simulink model "Detachable_Battery_Pack_V2"  (R2024a)
settings: Solver=VariableStepAuto  StartTime=0.0  StopTime=3600*2  RelTol=1e-3
libraries: fl_lib x5, nesl_utility x3, simulink x2, batt_lib x1, BatteryPack_UR18650ZTA_lib x1
settings Model: Creator=MANSY  LastModifiedBy=MANSY

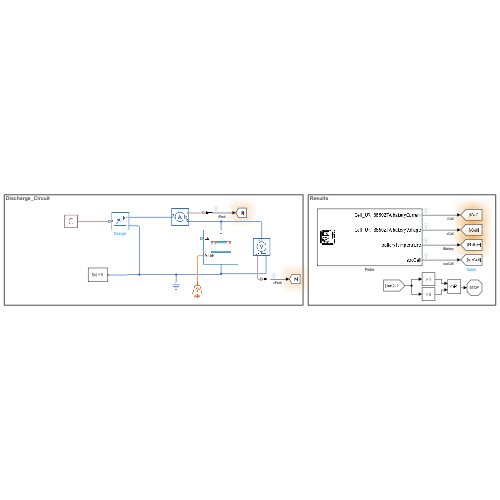
[thumbnail: Simulink's stored preview of the top-level diagram]
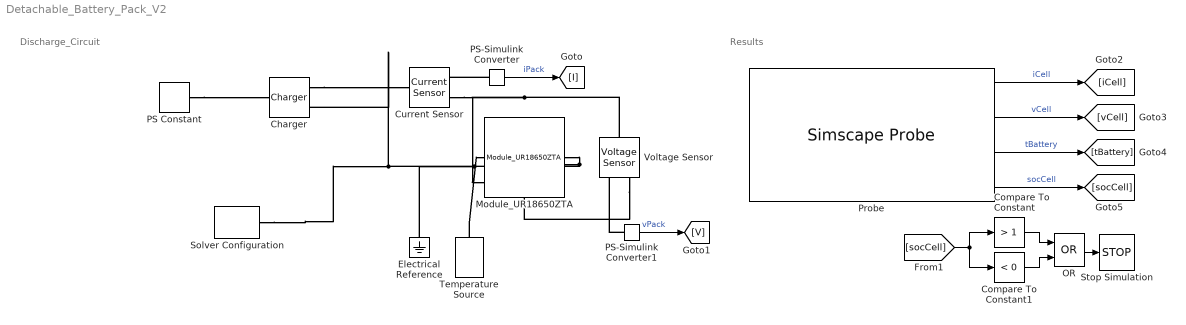
== system Detachable_Battery_Pack_V2 ==
  note: Results
  note: Discharge_Circuit
  Charger : batt_lib/Cyclers/Charger  charging_current=10.6 A  voltage_threshold=21 V  charging_voltage=21 V  current_threshold=0.5 A
      settings: InternalSimscapePortConfiguration="{\"Bottom\":[],\"Left\":[{\"id\":\"trigger\",\"label\":\"t\",\"type\":\"input\"}],\"Right\":[{\"id\":\"p\",\"label\":\"+\",\"type\":\"foundation.electrical.electrical\"},{\"id\":\"n\",\"label\":\"-\",\"type\":\"foundation.electrical.electrical\"}],\"Top\":[]}"
  Compare To Constant : simulink/Logic and Bit Operations/Compare To Constant  relop=>  const=1  OutDataTypeStr=boolean
  Compare To Constant1 : simulink/Logic and Bit Operations/Compare To Constant  relop=<  const=0  OutDataTypeStr=boolean
  Current Sensor : fl_lib/Electrical/Electrical Sensors/Current Sensor
  Electrical Reference : fl_lib/Electrical/Electrical Elements/Electrical Reference
  Module_UR18650ZTA : BatteryPack_UR18650ZTA_lib/Module_UR18650ZTA  BatteryCapacityCell=2.65 A*hr  ExtrapolationMethodCell=simscape.enum.extrapolation.linear  SOCBreakpointsCell=[0, .01, .02, .03, .04, .05, .06, .07, .08, .09, .1, .11, .12, .13, .14, .15, .16, .17, .18, .19, .2, .21, .22, .23, .24, .25, .26, .27, .28, .29, .3, .31, .32, .33, .34, .35, .36, .37, .38, .39, .4, .41, .42, .43, .44, .45, .46, .47, .48, .49, .5, .51, .52, .53, .54, .55, .56, .57, .58, .59, .6, .61, .62, .63, .64, .65, .66, .67, .68, .69, .7, .71, .72, .73, .74, .75, .76, .77, .78, .79, .8, .81, .82, .83, .84, .85, .86, .87, .88, .89, .9, .91, .92, .93, .94, .95, .96, .97, .98, .99, 1]  TemperatureBreakpointsCell=[0, 25, 40, 60] degC  OpenCircuitVoltageThermalCell=[3.04339, 3.04339, 3.04339, 3.04339; 3.19969, 3.19969, 3.19969, 3.19969; 3.32733, 3.32733, 3.32733, 3.32733; 3.41897, 3.41897, 3.41897, 3.41897; 3.47789, 3.47789, 3.47789, 3.47789; 3.5189, 3.5189, 3.5189, 3.5189; 3.54757, 3.54757, 3.54757, 3.54757; 3.56926, 3.56926, 3.56926, 3.56926; 3.58543, 3.58543, 3.58543, 3.58543; 3.59715, 3.59715, 3.59715, 3.59715; 3.60656, 3.60656, 3.60656, 3.60656; 3.61458, 3.61458, 3.61458, 3.61458; 3.62125, 3.62125, 3.62125, 3.62125; 3.62859, 3.62859, 3.62859, 3.62859; 3.63585, 3.63585, 3.63585, 3.63585; 3.64117, 3.64117, 3.64117, 3.64117; 3.64677, 3.64677, 3.64677, 3.64677; 3.65281, 3.65281, 3.65281, 3.65281; 3.65754, 3.65754, 3.65754, 3.65754; 3.6622, 3.6622, 3.6622, 3.6622; 3.66686, 3.66686, 3.66686, 3.66686; 3.67118, 3.67118, 3.67118, 3.67118; 3.67547, 3.67547, 3.67547, 3.67547; 3.67953, 3.67953, 3.67953, 3.67953; 3.68333, 3.68333, 3.68333, 3.68333; 3.68679, 3.68679, 3.68679, 3.68679; 3.68929, 3.68929, 3.68929, 3.68929; 3.69163, 3.69163, 3.69163, 3.69163; 3.69398, 3.69398, 3.69398, 3.69398; 3.69633, 3.69633, 3.69633, 3.69633; 3.69868, 3.69868, 3.69868, 3.69868; 3.70108, 3.70108, 3.70108, 3.70108; 3.7035, 3.7035, 3.7035, 3.7035; 3.70592, 3.70592, 3.70592, 3.70592; 3.70834, 3.70834, 3.70834, 3.70834; 3.71076, 3.71076, 3.71076, 3.71076; 3.71334, 3.71334, 3.71334, 3.71334; 3.71599, 3.71599, 3.71599, 3.71599; 3.71889, 3.71889, 3.71889, 3.71889; 3.72198, 3.72198, 3.72198, 3.72198; 3.72508, 3.72508, 3.72508, 3.72508; 3.72817, 3.72817, 3.72817, 3.72817; 3.73126, 3.73126, 3.73126, 3.73126; 3.73436, 3.73436, 3.73436, 3.73436; 3.73745, 3.73745, 3.73745, 3.73745; 3.74054, 3.74054, 3.74054, 3.74054; 3.74364, 3.74364, 3.74364, 3.74364; 3.74686, 3.74686, 3.74686, 3.74686; 3.75011, 3.75011, 3.75011, 3.75011; 3.75346, 3.75346, 3.75346, 3.75346; 3.75768, 3.75768, 3.75768, 3.75768; 3.7621, 3.7621, 3.7621, 3.7621; 3.76652, 3.76652, 3.76652, 3.76652; 3.77094, 3.77094, 3.77094, 3.77094; 3.77575, 3.77575, 3.77575, 3.77575; 3.78058, 3.78058, 3.78058, 3.78058; 3.78546, 3.78546, 3.78546, 3.78546; 3.79147, 3.79147, 3.79147, 3.79147; 3.79777, 3.79777, 3.79777, 3.79777; 3.80409, 3.80409, 3.80409, 3.80409; 3.8104, 3.8104, 3.8104, 3.8104; 3.81672, 3.81672, 3.81672, 3.81672; 3.82303, 3.82303, 3.82303, 3.82303; 3.82935, 3.82935, 3.82935, 3.82935; 3.83618, 3.83618, 3.83618, 3.83618; 3.84344, 3.84344, 3.84344, 3.84344; 3.8508, 3.8508, 3.8508, 3.8508; 3.85816, 3.85816, 3.85816, 3.85816; 3.86553, 3.86553, 3.86553, 3.86553; 3.87289, 3.87289, 3.87289, 3.87289; 3.88052, 3.88052, 3.88052, 3.88052; 3.88833, 3.88833, 3.88833, 3.88833; 3.89603, 3.89603, 3.89603, 3.89603; 3.90423, 3.90423, 3.90423, 3.90423; 3.91256, 3.91256, 3.91256, 3.91256; 3.92124, 3.92124, 3.92124, 3.92124; 3.93029, 3.93029, 3.93029, 3.93029; 3.93933, 3.93933, 3.93933, 3.93933; 3.94837, 3.94837, 3.94837, 3.94837; 3.95788, 3.95788, 3.95788, 3.95788; 3.96788, 3.96788, 3.96788, 3.96788; 3.97854, 3.97854, 3.97854, 3.97854; 3.98931, 3.98931, 3.98931, 3.98931; 4.00008, 4.00008, 4.00008, 4.00008; 4.01149, 4.01149, 4.01149, 4.01149; 4.02304, 4.02304, 4.02304, 4.02304; 4.03459, 4.03459, 4.03459, 4.03459; 4.04614, 4.04614, 4.04614, 4.04614; 4.05768, 4.05768, 4.05768, 4.05768; 4.06947, 4.06947, 4.06947, 4.06947; 4.08184, 4.08184, 4.08184, 4.08184; 4.09422, 4.09422, 4.09422, 4.09422; 4.1067, 4.1067, 4.1067, 4.1067; 4.11982, 4.11982, 4.11982, 4.11982; 4.1326, 4.1326, 4.1326, 4.1326; 4.14615, 4.14615, 4.14615, 4.14615; 4.15754, 4.15754, 4.15754, 4.15754; 4.16699, 4.16699, 4.16699, 4.16699; 4.17222, 4.17222, 4.17222, 4.17222; 4.18119, 4.18119, 4.18119, 4.18119; 4.30838, 4.30838, 4.30838, 4.30838] V  VoltageRangeCell=[2.7, Inf] V  ResistanceSOCBreakpointsCell=[0, .01, .02, .03, .04, .05, .06, .07, .08, .09, .1, .11, .12, .13, .14, .15, .16, .17, .18, .19, .2, .21, .22, .23, .24, .25, .26, .27, .28, .29, .3, .31, .32, .33, .34, .35, .36, .37, .38, .39, .4, .41, .42, .43, .44, .45, .46, .47, .48, .49, .5, .51, .52, .53, .54, .55, .56, .57, .58, .59, .6, .61, .62, .63, .64, .65, .66, .67, .68, .69, .7, .71, .72, .73, .74, .75, .76, .77, .78, .79, .8, .81, .82, .83, .84, .85, .86, .87, .88, .89, .9, .91, .92, .93, .94, .95, .96, .97, .98, .99, 1]  ResistanceTemperatureBreakpointsCell=[0, 25, 40, 60] degC  R0ThermalCell=[.10009, .04577, .01007, .01632; .14613, .0693, .01231, .013; .1823, .0871, .02576, .02712; .20605, .0981, .03749, .03657; .21852, .10274, .04624, .03593; .22481, .10473, .05239, .04275; .22685, .1047, .05724, .04532; .22648, .10401, .05969, .04893; .22421, .1029, .06023, .05216; .2204, .10084, .06022, .05386; .2158, .09855, .06061, .05477; .21072, .0961, .06053, .05519; .20518, .09374, .05997, .05515; .19986, .0923, .05976, .05534; .19452, .09098, .06051, .05551; .19005, .08942, .06059, .055; .18649, .08829, .06076, .05491; .18308, .08779, .06108, .05531; .17921, .08711, .06095, .05525; .17533, .08642, .06116, .05516; .17188, .08573, .06162, .05537; .16959, .08504, .06197, .05562; .16728, .08435, .0623, .05586; .16489, .08362, .06255, .05603; .16242, .08285, .06272, .0561; .15982, .0821, .06284, .05605; .15726, .08136, .06262, .05568; .15524, .08067, .06235, .05525; .15322, .07998, .06208, .05483; .1512, .07929, .06181, .05441; .14918, .07859, .06154, .05399; .14718, .07791, .06129, .05359; .14518, .07723, .06105, .05316; .14319, .07655, .06062, .05273; .14155, .07588, .06014, .0523; .14028, .0752, .05965, .05186; .13906, .07463, .05921, .05149; .13787, .07414, .0588, .05114; .13676, .07372, .05848, .05087; .13572, .07333, .05823, .05067; .13469, .07295, .05797, .05047; .13365, .07256, .05771, .05028; .13261, .07218, .05746, .0497; .13157, .07179, .0572, .04908; .13053, .07141, .05667, .04845; .12949, .07102, .05603, .04793; .1286, .07064, .05539, .04744; .12808, .07034, .05479, .04699; .12757, .07007, .0542, .04656; .1271, .06981, .05364, .04615; .12693, .06973, .05339, .04605; .12682, .0697, .0532, .04601; .12672, .06966, .05301, .04589; .12661, .06963, .05283, .04564; .12664, .06966, .05277, .04553; .12668, .06969, .05273, .04542; .12673, .06974, .0527, .04507; .12716, .07, .05306, .04491; .12758, .07016, .053, .04485; .128, .07032, .0529, .04479; .12841, .07047, .0528, .04474; .12883, .07062, .0527, .04468; .12925, .07078, .05261, .04463; .12967, .07093, .05251, .04457; .13027, .07117, .05259, .04469; .13101, .0715, .05282, .04497; .13204, .07186, .05308, .04484; .13321, .07221, .05335, .04472; .13439, .07256, .0532, .04459; .13557, .07292, .05301, .04446; .13684, .07332, .05292, .04443; .13817, .07375, .05288, .04428; .13946, .0741, .05281, .04407; .14091, .07448, .05291, .04404; .14233, .07489, .05306, .04405; .14388, .07535, .05333, .04418; .14556, .07584, .05372, .04444; .14723, .07633, .05411, .0447; .14891, .07682, .0545, .04496; .15108, .07759, .05506, .04537; .15372, .07866, .05578, .04596; .15659, .07988, .05673, .04678; .1595, .08112, .0574, .04703; .16241, .08236, .05796, .04728; .16616, .08368, .05874, .04774; .17134, .08499, .05957, .04825; .17651, .0863, .0604, .04877; .18169, .08761, .06123, .04928; .18774, .08891, .06206, .04979; .19646, .09039, .06297, .05038; .20538, .09225, .06408, .05118; .2143, .09411, .0652, .05198; .22836, .09597, .06593, .05281; .24309, .09796, .06644, .05348; .25899, .0995, .06683, .05394; .28056, .10104, .06749, .05466; .30009, .10043, .0674, .05464; .31508, .09826, .06607, .05332; .32861, .09216, .06054, .05002; .31916, .08512, .05631, .04686; .33322, .00997, .09284, .03396] Ohm  BatteryThermalMassCell=44.1 J/K  AmbientResistance=25 K/W  CellBalancingClosedResistance=0.01 Ohm  CellBalancingOpenConductance=1e-8 1/Ohm  CellBalancingThreshold=0.5  CellBalancingResistance=10 Ohm  P=4  S=5  socCell_specify=on  socCell_priority=High  socCell=0  socCell_nominal_specify=off  socCell_nominal_value=1  socCell_nominal_unit=1  numCycles_specify=off  numCycles_priority=High  numCycles=0  numCycles_nominal_specify=off  numCycles_nominal_value=1  numCycles_nominal_unit=1  batteryVoltage_specify=off  batteryVoltage_priority=None  batteryVoltage=0 V  batteryVoltage_nominal_specify=off  batteryVoltage_nominal_value=1  batteryVoltage_nominal_unit=V  batteryCurrent_specify=off  batteryCurrent_priority=None  batteryCurrent=0 A  batteryCurrent_nominal_specify=off  batteryCurrent_nominal_value=1  batteryCurrent_nominal_unit=A  batteryTemperature_specify=off  batteryTemperature_priority=High  batteryTemperature=298.15 K  batteryTemperature_nominal_specify=off  batteryTemperature_nominal_value=1  batteryTemperature_nominal_unit=K  vParallelAssembly_specify=off  vParallelAssembly_priority=None  vParallelAssembly=repmat(0, 5, 1) V  vParallelAssembly_nominal_specify=off  vParallelAssembly_nominal_value=1  vParallelAssembly_nominal_unit=V  socParallelAssembly_specify=off  socParallelAssembly_priority=None  socParallelAssembly=repmat(1, 5, 1)  socParallelAssembly_nominal_specify=off  socParallelAssembly_nominal_value=1  socParallelAssembly_nominal_unit=1
      settings: InternalSimscapePortConfiguration="{\"Bottom\":[{\"id\":\"n\",\"label\":\"-\",\"type\":\"foundation.electrical.electrical\"}],\"Left\":[{\"id\":\"enableCellBalancing\",\"label\":\"CB\",\"type\":\"input\"},{\"id\":\"AmbH\",\"label\":\"AmbH\",\"type\":\"foundation.thermal.thermal\"}],\"Right\":[],\"Top\":[{\"id\":\"p\",\"label\":\"+\",\"type\":\"foundation.electrical.electrical\"}]}"
  OR : Logic  Operator=OR  AllPortsSameDT=off  OutDataTypeStr=boolean
  PS Constant : fl_lib/Physical Signals/Sources/PS Constant  constant=1
  PS-Simulink Converter : nesl_utility/PS-Simulink Converter  PhysicalDomain=network_engine_domain  SubClassName=ps_output  LeftPortType=input  RightPortType=output  PseudoPeriodic=off  Frequencies=[]  VectorFormat=inherit  Unit=inherit  AffineConversion=off
  PS-Simulink Converter1 : nesl_utility/PS-Simulink Converter  PhysicalDomain=network_engine_domain  SubClassName=ps_output  LeftPortType=input  RightPortType=output  PseudoPeriodic=off  Frequencies=[]  VectorFormat=inherit  Unit=inherit  AffineConversion=off
  Probe : SimscapeProbe  BoundBlock=1  Variables={Cell_UR18650ZTA.batteryCurrent, Cell_UR18650ZTA.batteryVoltage, batteryTemperature, socCell}
  Solver Configuration : nesl_utility/Solver Configuration  PhysicalDomain=network_engine_domain  SubClassName=solver  LeftPortType=input  RightPortType=generic  Tones=[]  Harmonics=[]  SimulateNoise=off  Profile=off  UseLocalSampling=off  EnableSwitchedLinearOptims=on  FrequencyDomain=off  UseCCode=off  RelTol=0.001  AbsTol=0.001  MinStep=1e-09  ToWorkspace=off  RevertToSquareIcSolve=off  NumHomotopyIterations=100  PhasorMode=off  PhasorModeNumHarmonics=1  ConsistencySolver=NEWTON_XTOL_AFTER_FTOL  IndexReductionMethod=DerivativeReplacement  DoDC=off  ResidualTolerance=1e-09  ConsistencyTolSource=GLOBAL  ConsistencyAbsTol=0.001  ConsistencyRelTol=0.001  ConsistencyTolFactor=0.001  UseLocalSolver=off  LocalSolverChoice=NE_BACKWARD_EULER_ADVANCER  ResolveIndetEquations=on  FunctionEvalNumThread=1  LocalSolverSampleTime=0.001  DoFixedCost=off  MaxNonlinIter=3  MaxModeIter=2  ComputeImpulses=off  ImpulseIterations=2  LinearAlgebra=auto  LinearAlgebraNumThread=0  EquationFormulation=NE_TIME_EF  DelaysMemoryBudget=1024  AutomaticFiltering=on  FilteringTimeConstant=0.001  PartitionStorageMethod=AS_NEEDED  PartitionMemoryBudget=1024  PartitionMethod=ROBUST  MultibodyUseLocalSolver=off  MultibodyLocalSolverChoice=ODE1  MultibodyLocalSolverSampleTime=0.001
  Stop Simulation : Stop
  Temperature Source : fl_lib/Thermal/Thermal Sources/Temperature Source  temperature=295 K
  Voltage Sensor : fl_lib/Electrical/Electrical Sensors/Voltage Sensor
  wires:
  PS-Simulink Converter1/1 -> [V]  "vPack"
  PS-Simulink Converter/1 -> [I]  "iPack"
  Probe/2 -> [vCell]  "vCell"
  Probe/1 -> [iCell]  "iCell"
  Probe/3 -> [tBattery]  "tBattery"
  Probe/4 -> [socCell]  "socCell"
  OR/1 -> Stop Simulation/1
  Compare To Constant/1 -> OR/1
  Compare To Constant1/1 -> OR/2
  [socCell] -> Compare To Constant1/1, Compare To Constant/1
  connections:
  PS-Simulink Converter/LConn1 -- Current Sensor/RConn1
  Temperature Source/LConn1 -- Module_UR18650ZTA/LConn2
  PS-Simulink Converter1/LConn1 -- Voltage Sensor/RConn1
  Voltage Sensor/LConn1 -- Current Sensor/RConn2 -- Module_UR18650ZTA/LConn3
  Charger/RConn1 -- Current Sensor/LConn1
  Module_UR18650ZTA/RConn1 -- Voltage Sensor/RConn2 -- Electrical Reference/LConn1 -- Solver Configuration/RConn1 -- Charger/RConn2
  PS Constant/RConn1 -- Charger/LConn1
